simulink model "test_SimulinkMdl3LPV_Baseline"  (R2019b)
settings: Solver=FixedStepAuto  StartTime=0.0  StopTime=400  FixedStep=DT  RelTol=1e-3
values from neighbouring files (symbols this model uses):
  DT = 0.008    [dataDLR.m]    (also in generateReport.m; initLPVParam.m; initWorkspace.m; runCalculateEvalCriteria.m)
  Lin_points : value not decoded    [DD_test.sldd]
undefined symbols (not defined in the file or in its folder): Rotor_Lambda
settings Model: DataDictionary=DD_test.sldd  ExtModeTrigMode=oneshot  ExtModeArmWhenConnect=off  Creator=Hazim Namik  LastModifiedBy=ditt_aj
settings DataIOCC: LimitDataPoints=on  SaveFormat=Array  ReturnWorkspaceOutputs=off
settings OptimizationCC: BlockReduction=off  BooleanDataType=off  LifeSpan=inf
settings DebuggingCC: SaveWithParameterizedLinksMsg=none  UnderspecifiedInitializationDetection=Classic  MergeDetectMultiDrivingBlocksExec=none  SignalResolutionControl=TryResolveAllWithWarning  SFUnexpectedBacktrackingDiag=warning  SFNoUnconditionalDefaultTransitionDiag=warning  SFExecutionAtInitializationDiag=none  ArithmeticOperatorsInVariantConditions=warning
settings HardwareCC: ProdBitPerPointer=32  ProdBitPerSizeT=32  ProdBitPerPtrDiffT=32  ProdLargestAtomicFloat=None  ProdIntDivRoundTo=Undefined  ProdEndianess=Unspecified  ProdWordSize=32  ProdHWDeviceType=32-bit Generic  TargetUnknown=on
settings ModelReferenceCC: PropagateSignalLabelsOutOfModel=off
settings SFSimCC: SimUseLocalCustomCode=off  CustomCodeUndefinedFunction=UseInterfaceOnly
settings RTWCC: RTWUseLocalCustomCode=off
settings CodeAppCC: StateflowObjectComments=on
settings GRTTargetCC: TargetLangStandard=C89/C90 (ANSI)  GeneratePreprocessorConditionals=Disable all
settings ConfigComp: CovMetricSettings=dw  CovHtmlReporting=on  CovSaveCumulativeToWorkspaceVar=on  CovSaveSingleToWorkspaceVar=on  CovExternalEMLEnable=off

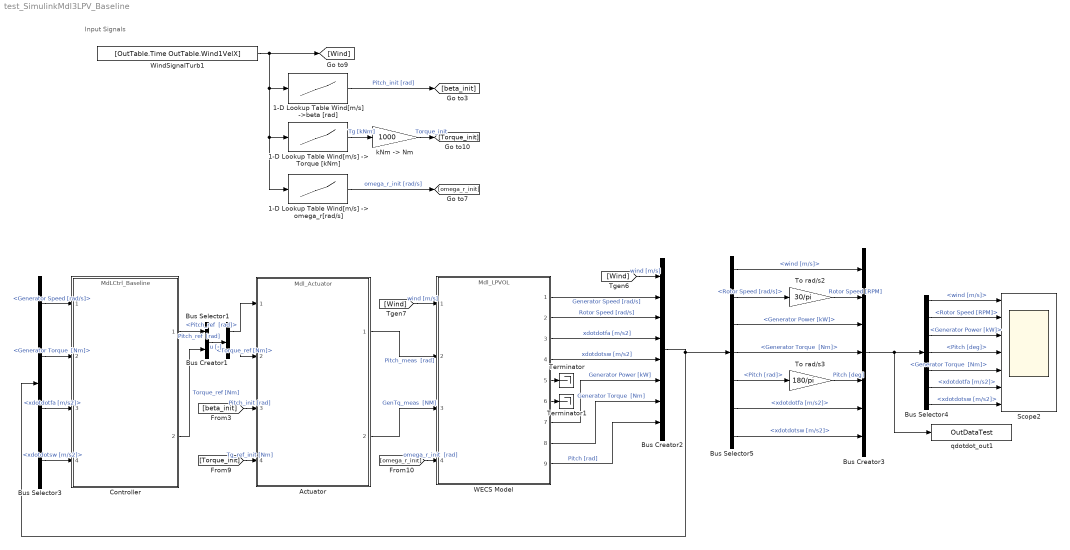
== system test_SimulinkMdl3LPV_Baseline ==
  note: Input Signals
  "1-D Lookup Table Wind[m/s] -> Torque [kNm]" : Lookup_n-D  NumberOfTableDimensions=1  BreakpointsForDimension1=Lin_points.V  BreakpointsForDimension2=Rotor_Lambda  Table=Lin_points.Torque  InternalRulePriority=Speed  RndMeth=Simplest  InputSameDT=on
  "1-D Lookup Table Wind[m/s] -> omega_r[rad/s]" : Lookup_n-D  NumberOfTableDimensions=1  BreakpointsForDimension1=Lin_points.V  BreakpointsForDimension2=Rotor_Lambda  Table=Lin_points.RSpeed  InternalRulePriority=Speed  RndMeth=Simplest  InputSameDT=on
  1-D Lookup Table Wind[m/s] ->beta [rad] : Lookup_n-D  NumberOfTableDimensions=1  BreakpointsForDimension1=Lin_points.V  BreakpointsForDimension2=Rotor_Lambda  Table=Lin_points.Pitch  InternalRulePriority=Speed  RndMeth=Simplest  InputSameDT=on
  Actuator : ModelReference  ModelNameDialog=Mdl_Actuator.slx  SimulationMode=Normal  ModelReferenceVersion=1.7
  Bus Creator1 : BusCreator  Inputs=2
  Bus Creator2 : BusCreator  Inputs=8
  Bus Creator3 : BusCreator  Inputs=7
  Bus Selector1 : BusSelector  OutputSignals="Pitch_ref  [rad],Torque_ref [Nm]"
  Bus Selector3 : BusSelector  OutputSignals="Generator Speed [rad/s],Generator Torque  [Nm],xdotdotfa [m/s2],xdotdotsw [m/s2]"
  Bus Selector4 : BusSelector  OutputSignals="wind [m/s],Rotor Speed [RPM],Generator Power [kW],Pitch [deg],Generator Torque  [Nm],xdotdotfa [m/s2],xdotdotsw [m/s2]"
  Bus Selector5 : BusSelector  OutputSignals="wind [m/s],Rotor Speed [rad/s],Generator Power [kW],Generator Torque  [Nm],Pitch [rad],xdotdotfa [m/s2],xdotdotsw [m/s2]"
  Controller : ModelReference  ModelNameDialog=MdLCtrl_Baseline.slx  SimulationMode=Normal  ModelReferenceVersion=1.13
  Scope2 : Scope  NumInputPorts=7
      settings: Tag=Scope
  Terminator : Terminator
  Terminator1 : Terminator
  To rad/s2 : Gain  Gain=30/pi
  To rad/s3 : Gain  Gain=180/pi
  WECS Model : ModelReference  ModelNameDialog=Mdl_LPVOL.slx  SimulationMode=Normal  ModelReferenceVersion=1.52
  WindSignalTurb1 : FromWorkspace  VariableName=[OutTable.Time OutTable.Wind1VelX]  SampleTime=DT  OutputAfterFinalValue=Holding final value
  "kNm -> Nm" : Gain  Gain=1000
  qdotdot_out1 : ToWorkspace  VariableName=OutDataTest  SampleTime=-1
  wires:
  Controller/2 -> Bus Creator1/2  "Torque_ref [Nm]"
  Bus Selector1/1 -> Actuator/1  "<Pitch_ref  [rad]>"
  [Torque_init] -> Actuator/4  "Tg_ref_init [Nm]"
  Bus Selector5/5 -> To rad/s3/1  "<Pitch [rad]>"
  WECS Model/6 -> Terminator1/1
  Bus Selector3/1 -> Controller/1  "<Generator Speed [rad/s]>"
  [omega_r_init] -> WECS Model/4  "omega_r_init  [rad]"
  Bus Creator2/1 -> Bus Selector3/1, Bus Selector5/1
  Actuator/2 -> WECS Model/3  "GenTq_meas  [NM]"
  WECS Model/5 -> Terminator/1
  [beta_init] -> Actuator/3  "Pitch_init [rad]"
  Bus Selector5/3 -> Bus Creator3/3  "<Generator Power [kW]>"
  "kNm -> Nm"/1 -> [Torque_init]  "Torque_init"
  Bus Selector3/4 -> Controller/4  "<xdotdotsw [m/s2]>"
  Bus Selector3/2 -> Controller/2  "<Generator Torque  [Nm]>"
  Bus Selector3/3 -> Controller/3  "<xdotdotfa [m/s2]>"
  To rad/s3/1 -> Bus Creator3/5  "Pitch [deg]"
  WindSignalTurb1/1 -> [Wind], "1-D Lookup Table Wind[m/s] -> omega_r[rad/s]"/1, "1-D Lookup Table Wind[m/s] -> Torque [kNm]"/1, 1-D Lookup Table Wind[m/s] ->beta [rad]/1
  Bus Selector5/4 -> Bus Creator3/4  "<Generator Torque  [Nm]>"
  Bus Selector5/2 -> To rad/s2/1  "<Rotor Speed [rad/s]>"
  Bus Selector5/6 -> Bus Creator3/6  "<xdotdotfa [m/s2]>"
  WECS Model/2 -> Bus Creator2/3  "Rotor Speed [rad/s]"
  [Wind] -> WECS Model/1  "wind [m/s]"
  Bus Selector4/3 -> Scope2/3  "<Generator Power [kW]>"
  "1-D Lookup Table Wind[m/s] -> Torque [kNm]"/1 -> "kNm -> Nm"/1  "Tg [kNm]"
  WECS Model/8 -> Bus Creator2/7  "Generator Torque  [Nm]"
  WECS Model/3 -> Bus Creator2/4  "xdotdotfa [m/s2]"
  1-D Lookup Table Wind[m/s] ->beta [rad]/1 -> [beta_init]  "Pitch_init [rad]"
  WECS Model/9 -> Bus Creator2/8  "Pitch [rad]"
  WECS Model/4 -> Bus Creator2/5  "xdotdotsw [m/s2]"
  "1-D Lookup Table Wind[m/s] -> omega_r[rad/s]"/1 -> [omega_r_init]  "omega_r_init [rad/s]"
  Bus Selector4/6 -> Scope2/6  "<xdotdotfa [m/s2]>"
  WECS Model/1 -> Bus Creator2/2  "Generator Speed [rad/s]"
  Controller/1 -> Bus Creator1/1  "Pitch_ref  [rad]"
  Bus Selector4/7 -> Scope2/7  "<xdotdotsw [m/s2]>"
  To rad/s2/1 -> Bus Creator3/2  "Rotor Speed [RPM]"
  [Wind] -> Bus Creator2/1  "wind [m/s]"
  Bus Selector1/2 -> Actuator/2  "<Torque_ref [Nm]>"
  Bus Selector4/4 -> Scope2/4  "<Pitch [deg]>"
  Bus Selector4/5 -> Scope2/5  "<Generator Torque  [Nm]>"
  Bus Selector4/1 -> Scope2/1  "<wind [m/s]>"
  Bus Selector4/2 -> Scope2/2  "<Rotor Speed [RPM]>"
  WECS Model/7 -> Bus Creator2/6  "Generator Power [kW]"
  Bus Selector5/1 -> Bus Creator3/1  "<wind [m/s]>"
  Actuator/1 -> WECS Model/2  "Pitch_meas  [rad]"
  Bus Selector5/7 -> Bus Creator3/7  "<xdotdotsw [m/s2]>"
  Bus Creator3/1 -> qdotdot_out1/1, Bus Selector4/1
  Bus Creator1/1 -> Bus Selector1/1  "u [-]"
